simulink model "RRTMS_Arsitektur_Fungsional"  (R2026a)
settings: Solver=VariableStepAuto
settings Model: Creator=afifah03  LastModifiedBy=afifah03

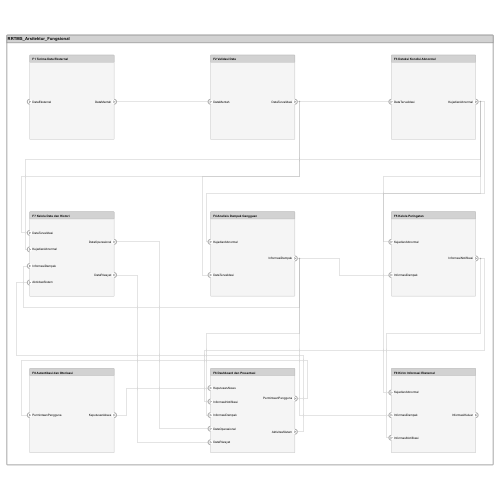
[thumbnail: Simulink's stored preview of the top-level diagram]
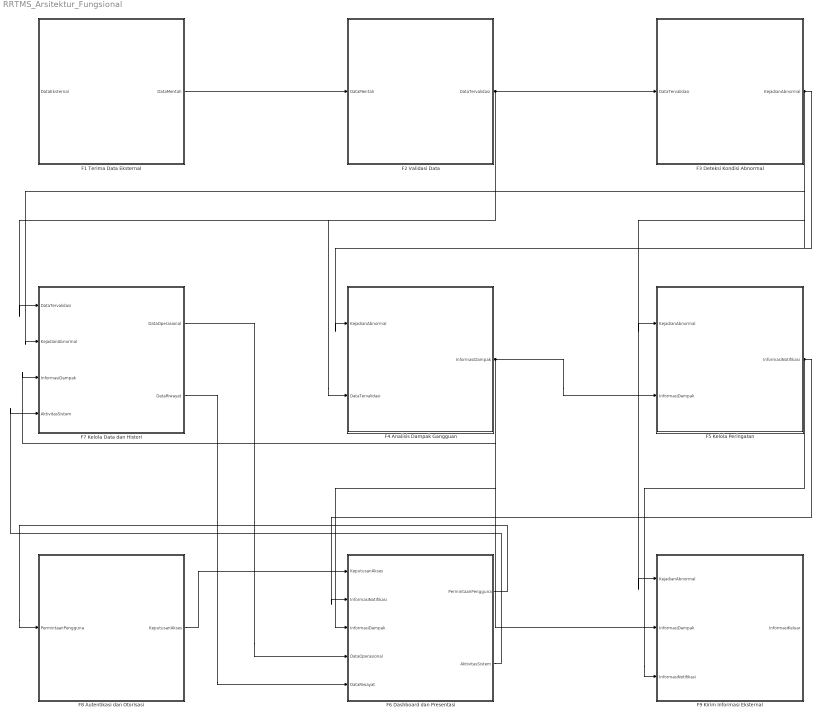
== system RRTMS_Arsitektur_Fungsional ==
  F1 Terima Data Eksternal : Subsystem
      settings: PortSchema="{\"entries\":[{\"content\":{\"headerSize\":26,\"margin\":15,\"minimumSpacing\":25,\"sides\":[{\"content\":{\"connectorIds\":[\"In1\"]},\"type\":\"ConnectorPlacement.EquallySpacedRectSide\",\"uuid\":\"944dc65e-47af-45ed-a139-0647cb5b290a\"},{\"content\":{\"connectorIds\":[\"Out1\"],\"side\":\"RIGHT\"},\"type\":\"ConnectorPlacement.EquallySpacedRectSide\",\"uuid\":\"cbdca632-76b6-4263-a090-790ed7d4bdf6\"},{\"content\":{\"side\":\"TOP\"},\"type\":\"ConnectorPlacement.EquallySpacedRectSide\",\"uuid\":\"9688978b-e9eb-4274-b3ec-2a343f050208\"}]},\"type\":\"ConnectorPlacement.EquallySpacedConnector\",\"uuid\":\"61d49fba-30a1-41fb-88c7-7b17ecf26b87\"}],\"packageUris\":[\"http://schema.mathworks.com/mf0/Connector/R2020b\"],\"version\":\"1.0\"}"
  F2 Validasi Data : Subsystem
      settings: PortSchema="{\"entries\":[{\"content\":{\"headerSize\":26,\"margin\":15,\"minimumSpacing\":25,\"sides\":[{\"content\":{\"connectorIds\":[\"In1\"]},\"type\":\"ConnectorPlacement.EquallySpacedRectSide\",\"uuid\":\"944dc65e-47af-45ed-a139-0647cb5b290a\"},{\"content\":{\"connectorIds\":[\"Out1\"],\"side\":\"RIGHT\"},\"type\":\"ConnectorPlacement.EquallySpacedRectSide\",\"uuid\":\"cbdca632-76b6-4263-a090-790ed7d4bdf6\"},{\"content\":{\"side\":\"TOP\"},\"type\":\"ConnectorPlacement.EquallySpacedRectSide\",\"uuid\":\"9688978b-e9eb-4274-b3ec-2a343f050208\"}]},\"type\":\"ConnectorPlacement.EquallySpacedConnector\",\"uuid\":\"61d49fba-30a1-41fb-88c7-7b17ecf26b87\"}],\"packageUris\":[\"http://schema.mathworks.com/mf0/Connector/R2020b\"],\"version\":\"1.0\"}"
  F3 Deteksi Kondisi Abnormal : Subsystem
      settings: PortSchema="{\"entries\":[{\"content\":{\"headerSize\":26,\"margin\":15,\"minimumSpacing\":25,\"sides\":[{\"content\":{\"connectorIds\":[\"In1\"]},\"type\":\"ConnectorPlacement.EquallySpacedRectSide\",\"uuid\":\"944dc65e-47af-45ed-a139-0647cb5b290a\"},{\"content\":{\"connectorIds\":[\"Out1\"],\"side\":\"RIGHT\"},\"type\":\"ConnectorPlacement.EquallySpacedRectSide\",\"uuid\":\"cbdca632-76b6-4263-a090-790ed7d4bdf6\"},{\"content\":{\"side\":\"TOP\"},\"type\":\"ConnectorPlacement.EquallySpacedRectSide\",\"uuid\":\"9688978b-e9eb-4274-b3ec-2a343f050208\"}]},\"type\":\"ConnectorPlacement.EquallySpacedConnector\",\"uuid\":\"61d49fba-30a1-41fb-88c7-7b17ecf26b87\"}],\"packageUris\":[\"http://schema.mathworks.com/mf0/Connector/R2020b\"],\"version\":\"1.0\"}"
  F4 Analisis Dampak Gangguan : Subsystem
      settings: PortSchema="{\"entries\":[{\"content\":{\"headerSize\":26,\"margin\":15,\"minimumSpacing\":25,\"sides\":[{\"content\":{\"connectorIds\":[\"In1\",\"In2\"]},\"type\":\"ConnectorPlacement.EquallySpacedRectSide\",\"uuid\":\"944dc65e-47af-45ed-a139-0647cb5b290a\"},{\"content\":{\"connectorIds\":[\"Out1\"],\"side\":\"RIGHT\"},\"type\":\"ConnectorPlacement.EquallySpacedRectSide\",\"uuid\":\"cbdca632-76b6-4263-a090-790ed7d4bdf6\"},{\"content\":{\"side\":\"TOP\"},\"type\":\"ConnectorPlacement.EquallySpacedRectSide\",\"uuid\":\"9688978b-e9eb-4274-b3ec-2a343f050208\"}]},\"type\":\"ConnectorPlacement.EquallySpacedConnector\",\"uuid\":\"61d49fba-30a1-41fb-88c7-7b17ecf26b87\"}],\"packageUris\":[\"http://schema.mathworks.com/mf0/Connector/R2020b\"],\"version\":\"1.0\"}"
  F5 Kelola Peringatan : Subsystem
      settings: PortSchema="{\"entries\":[{\"content\":{\"headerSize\":26,\"margin\":15,\"minimumSpacing\":25,\"sides\":[{\"content\":{\"connectorIds\":[\"In1\",\"In2\"]},\"type\":\"ConnectorPlacement.EquallySpacedRectSide\",\"uuid\":\"944dc65e-47af-45ed-a139-0647cb5b290a\"},{\"content\":{\"connectorIds\":[\"Out1\"],\"side\":\"RIGHT\"},\"type\":\"ConnectorPlacement.EquallySpacedRectSide\",\"uuid\":\"cbdca632-76b6-4263-a090-790ed7d4bdf6\"},{\"content\":{\"side\":\"TOP\"},\"type\":\"ConnectorPlacement.EquallySpacedRectSide\",\"uuid\":\"9688978b-e9eb-4274-b3ec-2a343f050208\"}]},\"type\":\"ConnectorPlacement.EquallySpacedConnector\",\"uuid\":\"61d49fba-30a1-41fb-88c7-7b17ecf26b87\"}],\"packageUris\":[\"http://schema.mathworks.com/mf0/Connector/R2020b\"],\"version\":\"1.0\"}"
  F6 Dashboard dan Presentasi : Subsystem
      settings: PortSchema="{\"entries\":[{\"content\":{\"headerSize\":26,\"margin\":15,\"minimumSpacing\":25,\"sides\":[{\"content\":{\"connectorIds\":[\"In1\",\"In2\",\"In3\",\"In4\",\"In5\"]},\"type\":\"ConnectorPlacement.EquallySpacedRectSide\",\"uuid\":\"944dc65e-47af-45ed-a139-0647cb5b290a\"},{\"content\":{\"connectorIds\":[\"Out1\",\"Out2\"],\"side\":\"RIGHT\"},\"type\":\"ConnectorPlacement.EquallySpacedRectSide\",\"uuid\":\"cbdca632-76b6-4263-a090-790ed7d4bdf6\"},{\"content\":{\"side\":\"TOP\"},\"type\":\"ConnectorPlacement.EquallySpacedRectSide\",\"uuid\":\"9688978b-e9eb-4274-b3ec-2a343f050208\"}]},\"type\":\"ConnectorPlacement.EquallySpacedConnector\",\"uuid\":\"61d49fba-30a1-41fb-88c7-7b17ecf26b87\"}],\"packageUris\":[\"http://schema.mathworks.com/mf0/Connector/R2020b\"],\"version\":\"1.0\"}"
  F7 Kelola Data dan Histori : Subsystem
      settings: PortSchema="{\"entries\":[{\"content\":{\"headerSize\":26,\"margin\":15,\"minimumSpacing\":25,\"sides\":[{\"content\":{\"connectorIds\":[\"In1\",\"In2\",\"In3\",\"In4\"]},\"type\":\"ConnectorPlacement.EquallySpacedRectSide\",\"uuid\":\"944dc65e-47af-45ed-a139-0647cb5b290a\"},{\"content\":{\"connectorIds\":[\"Out1\",\"Out2\"],\"side\":\"RIGHT\"},\"type\":\"ConnectorPlacement.EquallySpacedRectSide\",\"uuid\":\"cbdca632-76b6-4263-a090-790ed7d4bdf6\"},{\"content\":{\"side\":\"TOP\"},\"type\":\"ConnectorPlacement.EquallySpacedRectSide\",\"uuid\":\"9688978b-e9eb-4274-b3ec-2a343f050208\"}]},\"type\":\"ConnectorPlacement.EquallySpacedConnector\",\"uuid\":\"61d49fba-30a1-41fb-88c7-7b17ecf26b87\"}],\"packageUris\":[\"http://schema.mathworks.com/mf0/Connector/R2020b\"],\"version\":\"1.0\"}"
  F8 Autentikasi dan Otorisasi : Subsystem
      settings: PortSchema="{\"entries\":[{\"content\":{\"headerSize\":26,\"margin\":15,\"minimumSpacing\":25,\"sides\":[{\"content\":{\"connectorIds\":[\"In1\"]},\"type\":\"ConnectorPlacement.EquallySpacedRectSide\",\"uuid\":\"944dc65e-47af-45ed-a139-0647cb5b290a\"},{\"content\":{\"connectorIds\":[\"Out1\"],\"side\":\"RIGHT\"},\"type\":\"ConnectorPlacement.EquallySpacedRectSide\",\"uuid\":\"cbdca632-76b6-4263-a090-790ed7d4bdf6\"},{\"content\":{\"side\":\"TOP\"},\"type\":\"ConnectorPlacement.EquallySpacedRectSide\",\"uuid\":\"9688978b-e9eb-4274-b3ec-2a343f050208\"}]},\"type\":\"ConnectorPlacement.EquallySpacedConnector\",\"uuid\":\"61d49fba-30a1-41fb-88c7-7b17ecf26b87\"}],\"packageUris\":[\"http://schema.mathworks.com/mf0/Connector/R2020b\"],\"version\":\"1.0\"}"
  F9 Kirim Informasi Eksternal : Subsystem
      settings: PortSchema="{\"entries\":[{\"content\":{\"headerSize\":26,\"margin\":15,\"minimumSpacing\":25,\"sides\":[{\"content\":{\"connectorIds\":[\"In1\",\"In2\",\"In3\"]},\"type\":\"ConnectorPlacement.EquallySpacedRectSide\",\"uuid\":\"944dc65e-47af-45ed-a139-0647cb5b290a\"},{\"content\":{\"connectorIds\":[\"Out1\"],\"side\":\"RIGHT\"},\"type\":\"ConnectorPlacement.EquallySpacedRectSide\",\"uuid\":\"cbdca632-76b6-4263-a090-790ed7d4bdf6\"},{\"content\":{\"side\":\"TOP\"},\"type\":\"ConnectorPlacement.EquallySpacedRectSide\",\"uuid\":\"9688978b-e9eb-4274-b3ec-2a343f050208\"}]},\"type\":\"ConnectorPlacement.EquallySpacedConnector\",\"uuid\":\"61d49fba-30a1-41fb-88c7-7b17ecf26b87\"}],\"packageUris\":[\"http://schema.mathworks.com/mf0/Connector/R2020b\"],\"version\":\"1.0\"}"
  wires:
  F1 Terima Data Eksternal/1(DataMentah) -> F2 Validasi Data/1(DataMentah)
  F2 Validasi Data/1(DataTervalidasi) -> F3 Deteksi Kondisi Abnormal/1(DataTervalidasi), F4 Analisis Dampak Gangguan/2(DataTervalidasi), F7 Kelola Data dan Histori/1(DataTervalidasi)
  F3 Deteksi Kondisi Abnormal/1(KejadianAbnormal) -> F4 Analisis Dampak Gangguan/1(KejadianAbnormal), F5 Kelola Peringatan/1(KejadianAbnormal), F7 Kelola Data dan Histori/2(KejadianAbnormal), F9 Kirim Informasi Eksternal/1(KejadianAbnormal)
  F4 Analisis Dampak Gangguan/1(InformasiDampak) -> F5 Kelola Peringatan/2(InformasiDampak), F6 Dashboard dan Presentasi/3(InformasiDampak), F7 Kelola Data dan Histori/3(InformasiDampak), F9 Kirim Informasi Eksternal/2(InformasiDampak)
  F5 Kelola Peringatan/1(InformasiNotifikasi) -> F6 Dashboard dan Presentasi/2(InformasiNotifikasi), F9 Kirim Informasi Eksternal/3(InformasiNotifikasi)
  F7 Kelola Data dan Histori/1(DataOperasional) -> F6 Dashboard dan Presentasi/4(DataOperasional)
  F7 Kelola Data dan Histori/2(DataRiwayat) -> F6 Dashboard dan Presentasi/5(DataRiwayat)
  F6 Dashboard dan Presentasi/1(PermintaanPengguna) -> F8 Autentikasi dan Otorisasi/1(PermintaanPengguna)
  F8 Autentikasi dan Otorisasi/1(KeputusanAkses) -> F6 Dashboard dan Presentasi/1(KeputusanAkses)
  F6 Dashboard dan Presentasi/2(AktivitasSistem) -> F7 Kelola Data dan Histori/4(AktivitasSistem)

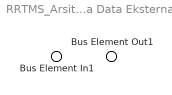
== system RRTMS_Arsitektur_Fungsional/F1 Terima Data Eksternal ==
  Bus Element In1 : Inport  PortName=DataEksternal
  Bus Element Out1 : Outport  PortName=DataMentah

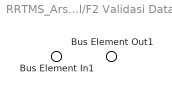
== system RRTMS_Arsitektur_Fungsional/F2 Validasi Data ==
  Bus Element In1 : Inport  PortName=DataMentah
  Bus Element Out1 : Outport  PortName=DataTervalidasi

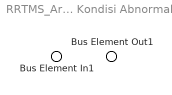
== system RRTMS_Arsitektur_Fungsional/F3 Deteksi Kondisi Abnormal ==
  Bus Element In1 : Inport  PortName=DataTervalidasi
  Bus Element Out1 : Outport  PortName=KejadianAbnormal

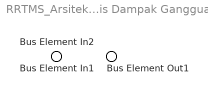
== system RRTMS_Arsitektur_Fungsional/F4 Analisis Dampak Gangguan ==
  Bus Element In1 : Inport  PortName=KejadianAbnormal
  Bus Element In2 : Inport  Port=2  PortName=DataTervalidasi
  Bus Element Out1 : Outport  PortName=InformasiDampak

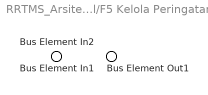
== system RRTMS_Arsitektur_Fungsional/F5 Kelola Peringatan ==
  Bus Element In1 : Inport  PortName=KejadianAbnormal
  Bus Element In2 : Inport  Port=2  PortName=InformasiDampak
  Bus Element Out1 : Outport  PortName=InformasiNotifikasi

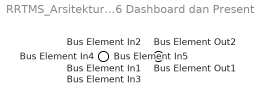
== system RRTMS_Arsitektur_Fungsional/F6 Dashboard dan Presentasi ==
  Bus Element In1 : Inport  PortName=KeputusanAkses
  Bus Element In2 : Inport  Port=2  PortName=InformasiNotifikasi
  Bus Element In3 : Inport  Port=3  PortName=InformasiDampak
  Bus Element In4 : Inport  Port=4  PortName=DataOperasional
  Bus Element In5 : Inport  Port=5  PortName=DataRiwayat
  Bus Element Out1 : Outport  PortName=PermintaanPengguna
  Bus Element Out2 : Outport  Port=2  PortName=AktivitasSistem

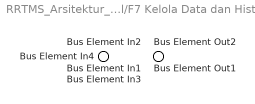
== system RRTMS_Arsitektur_Fungsional/F7 Kelola Data dan Histori ==
  Bus Element In1 : Inport  PortName=DataTervalidasi
  Bus Element In2 : Inport  Port=2  PortName=KejadianAbnormal
  Bus Element In3 : Inport  Port=3  PortName=InformasiDampak
  Bus Element In4 : Inport  Port=4  PortName=AktivitasSistem
  Bus Element Out1 : Outport  PortName=DataOperasional
  Bus Element Out2 : Outport  Port=2  PortName=DataRiwayat

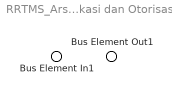
== system RRTMS_Arsitektur_Fungsional/F8 Autentikasi dan Otorisasi ==
  Bus Element In1 : Inport  PortName=PermintaanPengguna
  Bus Element Out1 : Outport  PortName=KeputusanAkses

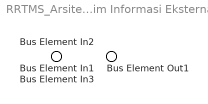
== system RRTMS_Arsitektur_Fungsional/F9 Kirim Informasi Eksternal ==
  Bus Element In1 : Inport  PortName=KejadianAbnormal
  Bus Element In2 : Inport  Port=2  PortName=InformasiDampak
  Bus Element In3 : Inport  Port=3  PortName=InformasiNotifikasi
  Bus Element Out1 : Outport  PortName=InformasiKeluar
